simulink model "bms_can_pack"  (R2026b)
settings: Solver=VariableStepAuto
undefined symbols (not defined in the file or in its folder): Ts
libraries: svdutilitieslib x7, simulink x1
settings Model: Creator=aomar  LastModifiedBy=aomar

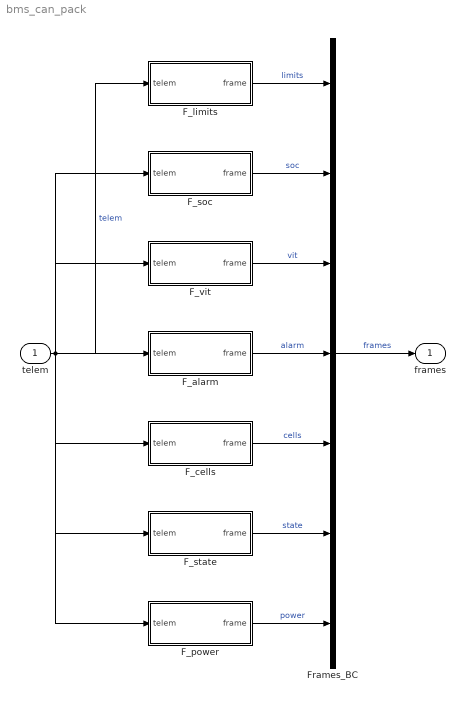
== system bms_can_pack ==
  telem : Inport  OutDataTypeStr=Bus: Bus_BMS_Telemetry  SampleTime=Ts.hk
  F_alarm : Subsystem
  F_cells : Subsystem
  F_limits : Subsystem
  F_power : Subsystem
  F_soc : Subsystem
  F_state : Subsystem
  F_vit : Subsystem
  Frames_BC : BusCreator  Inputs=7  OutDataTypeStr=Bus: Bus_Can1_Bms  NonVirtualBus=on
      settings: InheritFromInputs=off
  frames : Outport  OutDataTypeStr=Bus: Bus_Can1_Bms
  wires:
  telem/1 -> F_limits/1(telem), F_power/1(telem), F_soc/1(telem), F_state/1(telem), F_vit/1(telem), F_cells/1(telem), F_alarm/1(telem)  "telem"
  F_limits/1(frame) -> Frames_BC/1  "limits"
  F_soc/1(frame) -> Frames_BC/2  "soc"
  F_vit/1(frame) -> Frames_BC/3  "vit"
  F_alarm/1(frame) -> Frames_BC/4  "alarm"
  F_cells/1(frame) -> Frames_BC/5  "cells"
  F_state/1(frame) -> Frames_BC/6  "state"
  F_power/1(frame) -> Frames_BC/7  "power"
  Frames_BC/1 -> frames/1  "frames"

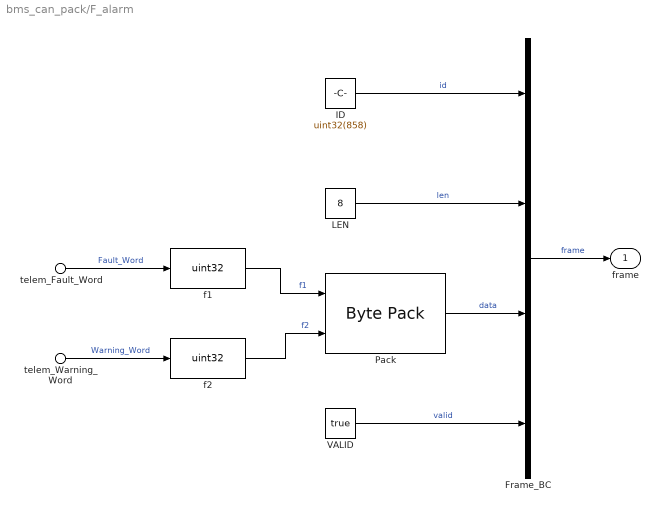
== system bms_can_pack/F_alarm ==
  telem_Fault_Word : Inport  PortName=telem  Element=Fault_Word
  telem_Warning_Word : Inport  PortName=telem  Element=Warning_Word
  Frame_BC : BusCreator  Inputs=4  OutDataTypeStr=Bus: Bus_CanFrame8  NonVirtualBus=on
      settings: InheritFromInputs=off
  ID : Constant  Value=uint32(858)  OutDataTypeStr=uint32  SampleTime=Ts.hk
  LEN : Constant  Value=8  OutDataTypeStr=uint8  SampleTime=Ts.hk
  Pack : svdutilitieslib/Byte Pack  maskPackedDataType=uint8  datatypes={'uint32','uint32'}  byteAlign=1  blockPlatform=arduinoert
      settings: LibrarySourceBlock=mcblib/Signal Management/Byte Pack
  VALID : Constant  Value=true  OutDataTypeStr=boolean  SampleTime=Ts.hk
  f1 : DataTypeConversion  OutDataTypeStr=uint32  RndMeth=Nearest
  f2 : DataTypeConversion  OutDataTypeStr=uint32  RndMeth=Nearest
  frame : Outport  OutDataTypeStr=Bus: Bus_CanFrame8
  wires:
  telem_Fault_Word/1 -> f1/1  "Fault_Word"
  telem_Warning_Word/1 -> f2/1  "Warning_Word"
  f1/1 -> Pack/1  "f1"
  f2/1 -> Pack/2  "f2"
  ID/1 -> Frame_BC/1  "id"
  LEN/1 -> Frame_BC/2  "len"
  VALID/1 -> Frame_BC/4  "valid"
  Pack/1 -> Frame_BC/3  "data"
  Frame_BC/1 -> frame/1  "frame"

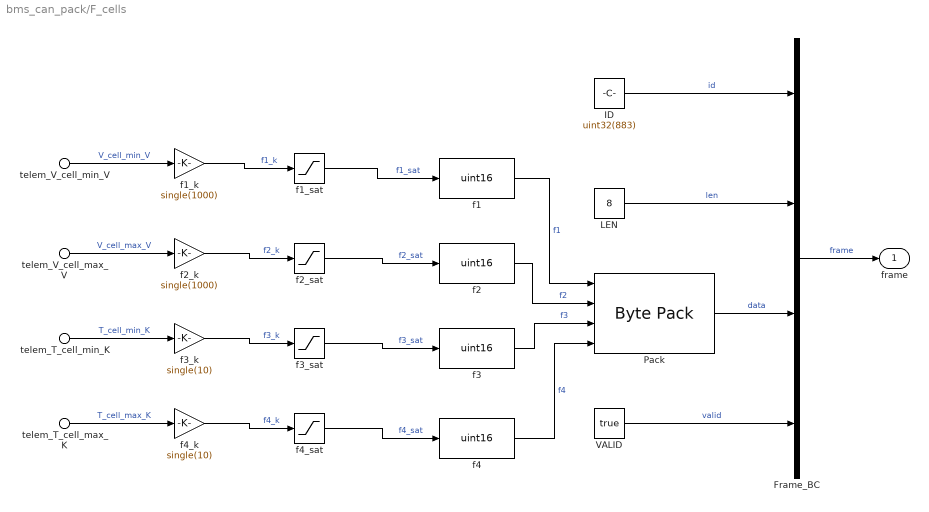
== system bms_can_pack/F_cells ==
  telem_V_cell_min_V : Inport  PortName=telem  Element=V_cell_min_V
  telem_V_cell_max_V : Inport  PortName=telem  Element=V_cell_max_V
  telem_T_cell_min_K : Inport  PortName=telem  Element=T_cell_min_K
  telem_T_cell_max_K : Inport  PortName=telem  Element=T_cell_max_K
  Frame_BC : BusCreator  Inputs=4  OutDataTypeStr=Bus: Bus_CanFrame8  NonVirtualBus=on
      settings: InheritFromInputs=off
  ID : Constant  Value=uint32(883)  OutDataTypeStr=uint32  SampleTime=Ts.hk
  LEN : Constant  Value=8  OutDataTypeStr=uint8  SampleTime=Ts.hk
  Pack : svdutilitieslib/Byte Pack  maskPackedDataType=uint8  datatypes={'uint16','uint16','uint16','uint16'}  byteAlign=1  blockPlatform=arduinoert
      settings: LibrarySourceBlock=mcblib/Signal Management/Byte Pack
  VALID : Constant  Value=true  OutDataTypeStr=boolean  SampleTime=Ts.hk
  f{1..4} (4 alike) : DataTypeConversion  OutDataTypeStr=uint16  RndMeth=Nearest
  f1_k : Gain  Gain=single(1000)
  f1_sat : Saturate  UpperLimit=single(intmax('uint16'))  LowerLimit=single(intmin('uint16'))
  f2_k : Gain  Gain=single(1000)
  f2_sat : Saturate  UpperLimit=single(intmax('uint16'))  LowerLimit=single(intmin('uint16'))
  f3_k : Gain  Gain=single(10)
  f3_sat : Saturate  UpperLimit=single(intmax('uint16'))  LowerLimit=single(intmin('uint16'))
  f4_k : Gain  Gain=single(10)
  f4_sat : Saturate  UpperLimit=single(intmax('uint16'))  LowerLimit=single(intmin('uint16'))
  frame : Outport  OutDataTypeStr=Bus: Bus_CanFrame8
  wires:
  telem_V_cell_min_V/1 -> f1_k/1  "V_cell_min_V"
  telem_V_cell_max_V/1 -> f2_k/1  "V_cell_max_V"
  telem_T_cell_min_K/1 -> f3_k/1  "T_cell_min_K"
  telem_T_cell_max_K/1 -> f4_k/1  "T_cell_max_K"
  f1_k/1 -> f1_sat/1  "f1_k"
  f2_k/1 -> f2_sat/1  "f2_k"
  f3_k/1 -> f3_sat/1  "f3_k"
  f4_k/1 -> f4_sat/1  "f4_k"
  f1_sat/1 -> f1/1  "f1_sat"
  f2_sat/1 -> f2/1  "f2_sat"
  f3_sat/1 -> f3/1  "f3_sat"
  f4_sat/1 -> f4/1  "f4_sat"
  f1/1 -> Pack/1  "f1"
  f2/1 -> Pack/2  "f2"
  f3/1 -> Pack/3  "f3"
  f4/1 -> Pack/4  "f4"
  ID/1 -> Frame_BC/1  "id"
  LEN/1 -> Frame_BC/2  "len"
  VALID/1 -> Frame_BC/4  "valid"
  Pack/1 -> Frame_BC/3  "data"
  Frame_BC/1 -> frame/1  "frame"

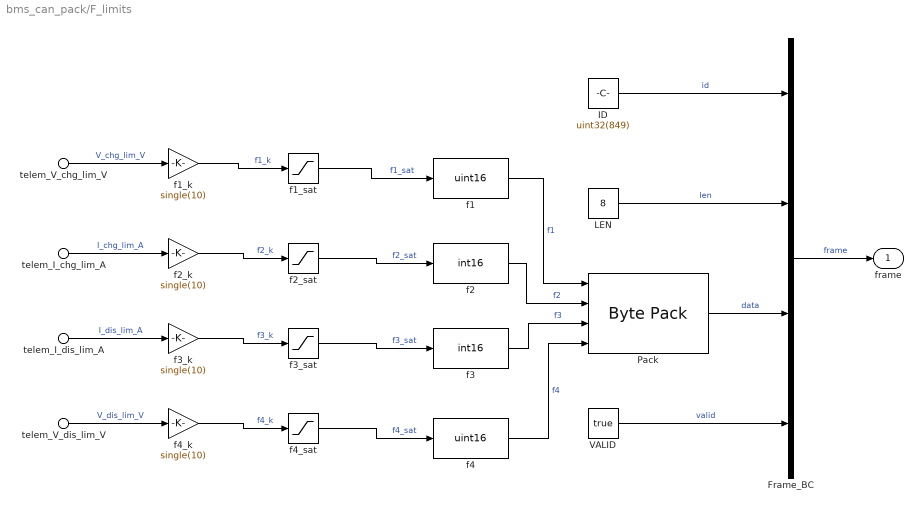
== system bms_can_pack/F_limits ==
  telem_V_chg_lim_V : Inport  PortName=telem  Element=V_chg_lim_V
  telem_I_chg_lim_A : Inport  PortName=telem  Element=I_chg_lim_A
  telem_I_dis_lim_A : Inport  PortName=telem  Element=I_dis_lim_A
  telem_V_dis_lim_V : Inport  PortName=telem  Element=V_dis_lim_V
  Frame_BC : BusCreator  Inputs=4  OutDataTypeStr=Bus: Bus_CanFrame8  NonVirtualBus=on
      settings: InheritFromInputs=off
  ID : Constant  Value=uint32(849)  OutDataTypeStr=uint32  SampleTime=Ts.hk
  LEN : Constant  Value=8  OutDataTypeStr=uint8  SampleTime=Ts.hk
  Pack : svdutilitieslib/Byte Pack  maskPackedDataType=uint8  datatypes={'uint16','int16','int16','uint16'}  byteAlign=1  blockPlatform=arduinoert
      settings: LibrarySourceBlock=mcblib/Signal Management/Byte Pack
  VALID : Constant  Value=true  OutDataTypeStr=boolean  SampleTime=Ts.hk
  f1 : DataTypeConversion  OutDataTypeStr=uint16  RndMeth=Nearest
  f1_k : Gain  Gain=single(10)
  f1_sat : Saturate  UpperLimit=single(intmax('uint16'))  LowerLimit=single(intmin('uint16'))
  f2 : DataTypeConversion  OutDataTypeStr=int16  RndMeth=Nearest
  f2_k : Gain  Gain=single(10)
  f2_sat : Saturate  UpperLimit=single(intmax('int16'))  LowerLimit=single(intmin('int16'))
  f3 : DataTypeConversion  OutDataTypeStr=int16  RndMeth=Nearest
  f3_k : Gain  Gain=single(10)
  f3_sat : Saturate  UpperLimit=single(intmax('int16'))  LowerLimit=single(intmin('int16'))
  f4 : DataTypeConversion  OutDataTypeStr=uint16  RndMeth=Nearest
  f4_k : Gain  Gain=single(10)
  f4_sat : Saturate  UpperLimit=single(intmax('uint16'))  LowerLimit=single(intmin('uint16'))
  frame : Outport  OutDataTypeStr=Bus: Bus_CanFrame8
  wires:
  telem_V_chg_lim_V/1 -> f1_k/1  "V_chg_lim_V"
  telem_I_chg_lim_A/1 -> f2_k/1  "I_chg_lim_A"
  telem_I_dis_lim_A/1 -> f3_k/1  "I_dis_lim_A"
  telem_V_dis_lim_V/1 -> f4_k/1  "V_dis_lim_V"
  f1_k/1 -> f1_sat/1  "f1_k"
  f2_k/1 -> f2_sat/1  "f2_k"
  f3_k/1 -> f3_sat/1  "f3_k"
  f4_k/1 -> f4_sat/1  "f4_k"
  f1_sat/1 -> f1/1  "f1_sat"
  f2_sat/1 -> f2/1  "f2_sat"
  f3_sat/1 -> f3/1  "f3_sat"
  f4_sat/1 -> f4/1  "f4_sat"
  f1/1 -> Pack/1  "f1"
  f2/1 -> Pack/2  "f2"
  f3/1 -> Pack/3  "f3"
  f4/1 -> Pack/4  "f4"
  ID/1 -> Frame_BC/1  "id"
  LEN/1 -> Frame_BC/2  "len"
  VALID/1 -> Frame_BC/4  "valid"
  Pack/1 -> Frame_BC/3  "data"
  Frame_BC/1 -> frame/1  "frame"

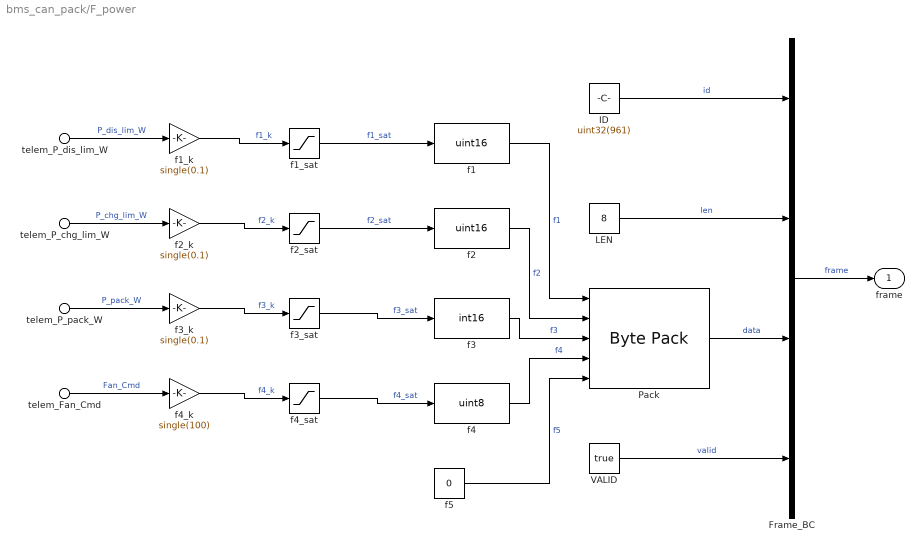
== system bms_can_pack/F_power ==
  telem_P_dis_lim_W : Inport  PortName=telem  Element=P_dis_lim_W
  telem_P_chg_lim_W : Inport  PortName=telem  Element=P_chg_lim_W
  telem_P_pack_W : Inport  PortName=telem  Element=P_pack_W
  telem_Fan_Cmd : Inport  PortName=telem  Element=Fan_Cmd
  Frame_BC : BusCreator  Inputs=4  OutDataTypeStr=Bus: Bus_CanFrame8  NonVirtualBus=on
      settings: InheritFromInputs=off
  ID : Constant  Value=uint32(961)  OutDataTypeStr=uint32  SampleTime=Ts.hk
  LEN : Constant  Value=8  OutDataTypeStr=uint8  SampleTime=Ts.hk
  Pack : svdutilitieslib/Byte Pack  maskPackedDataType=uint8  datatypes={'uint16','uint16','int16','uint8','uint8'}  byteAlign=1  blockPlatform=arduinoert
      settings: LibrarySourceBlock=mcblib/Signal Management/Byte Pack
  VALID : Constant  Value=true  OutDataTypeStr=boolean  SampleTime=Ts.hk
  f1 : DataTypeConversion  OutDataTypeStr=uint16  RndMeth=Nearest
  f1_k : Gain  Gain=single(0.1)
  f1_sat : Saturate  UpperLimit=single(intmax('uint16'))  LowerLimit=single(intmin('uint16'))
  f2 : DataTypeConversion  OutDataTypeStr=uint16  RndMeth=Nearest
  f2_k : Gain  Gain=single(0.1)
  f2_sat : Saturate  UpperLimit=single(intmax('uint16'))  LowerLimit=single(intmin('uint16'))
  f3 : DataTypeConversion  OutDataTypeStr=int16  RndMeth=Nearest
  f3_k : Gain  Gain=single(0.1)
  f3_sat : Saturate  UpperLimit=single(intmax('int16'))  LowerLimit=single(intmin('int16'))
  f4 : DataTypeConversion  OutDataTypeStr=uint8  RndMeth=Nearest
  f4_k : Gain  Gain=single(100)
  f4_sat : Saturate  UpperLimit=single(intmax('uint8'))  LowerLimit=single(intmin('uint8'))
  f5 : Constant  Value=0  OutDataTypeStr=uint8  SampleTime=Ts.hk
  frame : Outport  OutDataTypeStr=Bus: Bus_CanFrame8
  wires:
  telem_P_dis_lim_W/1 -> f1_k/1  "P_dis_lim_W"
  telem_P_chg_lim_W/1 -> f2_k/1  "P_chg_lim_W"
  telem_P_pack_W/1 -> f3_k/1  "P_pack_W"
  telem_Fan_Cmd/1 -> f4_k/1  "Fan_Cmd"
  f1_k/1 -> f1_sat/1  "f1_k"
  f2_k/1 -> f2_sat/1  "f2_k"
  f3_k/1 -> f3_sat/1  "f3_k"
  f4_k/1 -> f4_sat/1  "f4_k"
  f1_sat/1 -> f1/1  "f1_sat"
  f2_sat/1 -> f2/1  "f2_sat"
  f3_sat/1 -> f3/1  "f3_sat"
  f4_sat/1 -> f4/1  "f4_sat"
  f5/1 -> Pack/5  "f5"
  f1/1 -> Pack/1  "f1"
  f2/1 -> Pack/2  "f2"
  f3/1 -> Pack/3  "f3"
  f4/1 -> Pack/4  "f4"
  ID/1 -> Frame_BC/1  "id"
  LEN/1 -> Frame_BC/2  "len"
  VALID/1 -> Frame_BC/4  "valid"
  Pack/1 -> Frame_BC/3  "data"
  Frame_BC/1 -> frame/1  "frame"

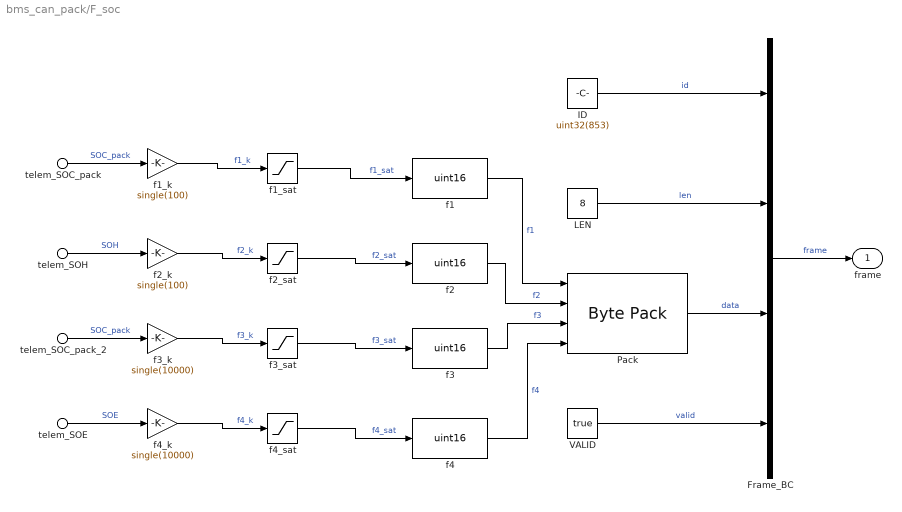
== system bms_can_pack/F_soc ==
  telem_SOC_pack : Inport  PortName=telem  Element=SOC_pack
  telem_SOC_pack_2 : Inport  PortName=telem  Element=SOC_pack
  telem_SOH : Inport  PortName=telem  Element=SOH
  telem_SOE : Inport  PortName=telem  Element=SOE
  Frame_BC : BusCreator  Inputs=4  OutDataTypeStr=Bus: Bus_CanFrame8  NonVirtualBus=on
      settings: InheritFromInputs=off
  ID : Constant  Value=uint32(853)  OutDataTypeStr=uint32  SampleTime=Ts.hk
  LEN : Constant  Value=8  OutDataTypeStr=uint8  SampleTime=Ts.hk
  Pack : svdutilitieslib/Byte Pack  maskPackedDataType=uint8  datatypes={'uint16','uint16','uint16','uint16'}  byteAlign=1  blockPlatform=arduinoert
      settings: LibrarySourceBlock=mcblib/Signal Management/Byte Pack
  VALID : Constant  Value=true  OutDataTypeStr=boolean  SampleTime=Ts.hk
  f{1..4} (4 alike) : DataTypeConversion  OutDataTypeStr=uint16  RndMeth=Nearest
  f1_k : Gain  Gain=single(100)
  f1_sat : Saturate  UpperLimit=single(intmax('uint16'))  LowerLimit=single(intmin('uint16'))
  f2_k : Gain  Gain=single(100)
  f2_sat : Saturate  UpperLimit=single(intmax('uint16'))  LowerLimit=single(intmin('uint16'))
  f3_k : Gain  Gain=single(10000)
  f3_sat : Saturate  UpperLimit=single(intmax('uint16'))  LowerLimit=single(intmin('uint16'))
  f4_k : Gain  Gain=single(10000)
  f4_sat : Saturate  UpperLimit=single(intmax('uint16'))  LowerLimit=single(intmin('uint16'))
  frame : Outport  OutDataTypeStr=Bus: Bus_CanFrame8
  wires:
  telem_SOC_pack/1 -> f1_k/1  "SOC_pack"
  telem_SOH/1 -> f2_k/1  "SOH"
  telem_SOC_pack_2/1 -> f3_k/1  "SOC_pack"
  telem_SOE/1 -> f4_k/1  "SOE"
  f1_k/1 -> f1_sat/1  "f1_k"
  f2_k/1 -> f2_sat/1  "f2_k"
  f3_k/1 -> f3_sat/1  "f3_k"
  f4_k/1 -> f4_sat/1  "f4_k"
  f1_sat/1 -> f1/1  "f1_sat"
  f2_sat/1 -> f2/1  "f2_sat"
  f3_sat/1 -> f3/1  "f3_sat"
  f4_sat/1 -> f4/1  "f4_sat"
  f1/1 -> Pack/1  "f1"
  f2/1 -> Pack/2  "f2"
  f3/1 -> Pack/3  "f3"
  f4/1 -> Pack/4  "f4"
  ID/1 -> Frame_BC/1  "id"
  LEN/1 -> Frame_BC/2  "len"
  VALID/1 -> Frame_BC/4  "valid"
  Pack/1 -> Frame_BC/3  "data"
  Frame_BC/1 -> frame/1  "frame"

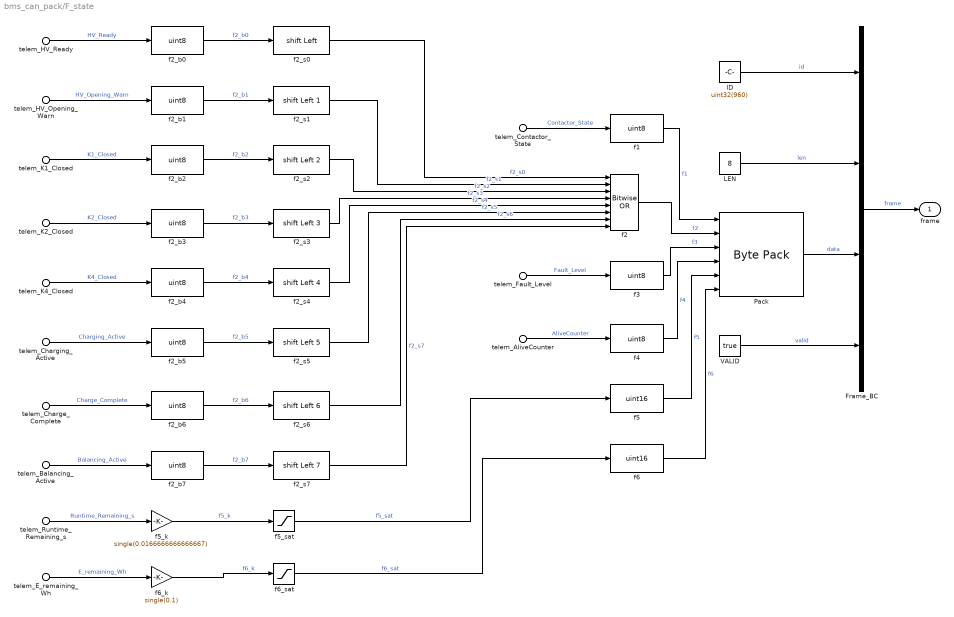
== system bms_can_pack/F_state ==
  telem_Contactor_State : Inport  PortName=telem  Element=Contactor_State
  telem_HV_Ready : Inport  PortName=telem  Element=HV_Ready
  telem_HV_Opening_Warn : Inport  PortName=telem  Element=HV_Opening_Warn
  telem_K1_Closed : Inport  PortName=telem  Element=K1_Closed
  telem_K2_Closed : Inport  PortName=telem  Element=K2_Closed
  telem_K4_Closed : Inport  PortName=telem  Element=K4_Closed
  telem_Charging_Active : Inport  PortName=telem  Element=Charging_Active
  telem_Charge_Complete : Inport  PortName=telem  Element=Charge_Complete
  telem_Balancing_Active : Inport  PortName=telem  Element=Balancing_Active
  telem_Fault_Level : Inport  PortName=telem  Element=Fault_Level
  telem_AliveCounter : Inport  PortName=telem  Element=AliveCounter
  telem_Runtime_Remaining_s : Inport  PortName=telem  Element=Runtime_Remaining_s
  telem_E_remaining_Wh : Inport  PortName=telem  Element=E_remaining_Wh
  Frame_BC : BusCreator  Inputs=4  OutDataTypeStr=Bus: Bus_CanFrame8  NonVirtualBus=on
      settings: InheritFromInputs=off
  ID : Constant  Value=uint32(960)  OutDataTypeStr=uint32  SampleTime=Ts.hk
  LEN : Constant  Value=8  OutDataTypeStr=uint8  SampleTime=Ts.hk
  Pack : svdutilitieslib/Byte Pack  maskPackedDataType=uint8  datatypes={'uint8','uint8','uint8','uint8','uint16','uint16'}  byteAlign=1  blockPlatform=arduinoert
      settings: LibrarySourceBlock=mcblib/Signal Management/Byte Pack
  VALID : Constant  Value=true  OutDataTypeStr=boolean  SampleTime=Ts.hk
  f1 : DataTypeConversion  OutDataTypeStr=uint8  RndMeth=Nearest
  f2 : simulink/Logic and Bit Operations/Bitwise Operator  logicop=OR  UseBitMask=off  NumInputPorts=8  BitMask=bin2dec('11011001')  BitMaskRealWorld=Stored Integer
  f2_b{0..7} (8 alike) : DataTypeConversion  OutDataTypeStr=uint8  RndMeth=Nearest
  f2_s0 : ArithShift  BitShiftDirection=Left
  f2_s1 : ArithShift  BitShiftNumber=1  BitShiftDirection=Left
  f2_s2 : ArithShift  BitShiftNumber=2  BitShiftDirection=Left
  f2_s3 : ArithShift  BitShiftNumber=3  BitShiftDirection=Left
  f2_s4 : ArithShift  BitShiftNumber=4  BitShiftDirection=Left
  f2_s5 : ArithShift  BitShiftNumber=5  BitShiftDirection=Left
  f2_s6 : ArithShift  BitShiftNumber=6  BitShiftDirection=Left
  f2_s7 : ArithShift  BitShiftNumber=7  BitShiftDirection=Left
  f3 : DataTypeConversion  OutDataTypeStr=uint8  RndMeth=Nearest
  f4 : DataTypeConversion  OutDataTypeStr=uint8  RndMeth=Nearest
  f5 : DataTypeConversion  OutDataTypeStr=uint16  RndMeth=Nearest
  f5_k : Gain  Gain=single(0.0166666666666667)
  f5_sat : Saturate  UpperLimit=single(intmax('uint16'))  LowerLimit=single(intmin('uint16'))
  f6 : DataTypeConversion  OutDataTypeStr=uint16  RndMeth=Nearest
  f6_k : Gain  Gain=single(0.1)
  f6_sat : Saturate  UpperLimit=single(intmax('uint16'))  LowerLimit=single(intmin('uint16'))
  frame : Outport  OutDataTypeStr=Bus: Bus_CanFrame8
  wires:
  telem_HV_Ready/1 -> f2_b0/1  "HV_Ready"
  telem_HV_Opening_Warn/1 -> f2_b1/1  "HV_Opening_Warn"
  telem_K1_Closed/1 -> f2_b2/1  "K1_Closed"
  telem_K2_Closed/1 -> f2_b3/1  "K2_Closed"
  telem_K4_Closed/1 -> f2_b4/1  "K4_Closed"
  telem_Charging_Active/1 -> f2_b5/1  "Charging_Active"
  telem_Charge_Complete/1 -> f2_b6/1  "Charge_Complete"
  telem_Balancing_Active/1 -> f2_b7/1  "Balancing_Active"
  telem_Runtime_Remaining_s/1 -> f5_k/1  "Runtime_Remaining_s"
  telem_E_remaining_Wh/1 -> f6_k/1  "E_remaining_Wh"
  f5_k/1 -> f5_sat/1  "f5_k"
  f6_k/1 -> f6_sat/1  "f6_k"
  f2_b0/1 -> f2_s0/1  "f2_b0"
  f2_b1/1 -> f2_s1/1  "f2_b1"
  f2_b2/1 -> f2_s2/1  "f2_b2"
  f2_b3/1 -> f2_s3/1  "f2_b3"
  f2_b4/1 -> f2_s4/1  "f2_b4"
  f2_b5/1 -> f2_s5/1  "f2_b5"
  f2_b6/1 -> f2_s6/1  "f2_b6"
  f2_b7/1 -> f2_s7/1  "f2_b7"
  f5_sat/1 -> f5/1  "f5_sat"
  f6_sat/1 -> f6/1  "f6_sat"
  f2_s0/1 -> f2/1  "f2_s0"
  f2_s1/1 -> f2/2  "f2_s1"
  f2_s2/1 -> f2/3  "f2_s2"
  f2_s3/1 -> f2/4  "f2_s3"
  f2_s4/1 -> f2/5  "f2_s4"
  f2_s5/1 -> f2/6  "f2_s5"
  f2_s6/1 -> f2/7  "f2_s6"
  f2_s7/1 -> f2/8  "f2_s7"
  telem_Contactor_State/1 -> f1/1  "Contactor_State"
  telem_Fault_Level/1 -> f3/1  "Fault_Level"
  telem_AliveCounter/1 -> f4/1  "AliveCounter"
  f2/1 -> Pack/2  "f2"
  f1/1 -> Pack/1  "f1"
  f3/1 -> Pack/3  "f3"
  f4/1 -> Pack/4  "f4"
  f5/1 -> Pack/5  "f5"
  f6/1 -> Pack/6  "f6"
  ID/1 -> Frame_BC/1  "id"
  LEN/1 -> Frame_BC/2  "len"
  VALID/1 -> Frame_BC/4  "valid"
  Pack/1 -> Frame_BC/3  "data"
  Frame_BC/1 -> frame/1  "frame"

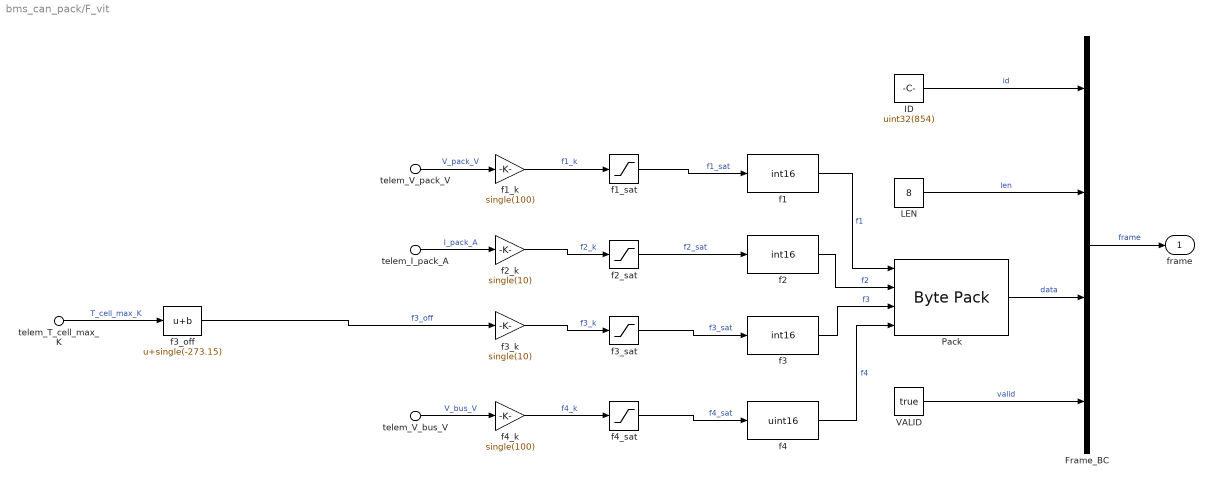
== system bms_can_pack/F_vit ==
  telem_V_pack_V : Inport  PortName=telem  Element=V_pack_V
  telem_I_pack_A : Inport  PortName=telem  Element=I_pack_A
  telem_T_cell_max_K : Inport  PortName=telem  Element=T_cell_max_K
  telem_V_bus_V : Inport  PortName=telem  Element=V_bus_V
  Frame_BC : BusCreator  Inputs=4  OutDataTypeStr=Bus: Bus_CanFrame8  NonVirtualBus=on
      settings: InheritFromInputs=off
  ID : Constant  Value=uint32(854)  OutDataTypeStr=uint32  SampleTime=Ts.hk
  LEN : Constant  Value=8  OutDataTypeStr=uint8  SampleTime=Ts.hk
  Pack : svdutilitieslib/Byte Pack  maskPackedDataType=uint8  datatypes={'int16','int16','int16','uint16'}  byteAlign=1  blockPlatform=arduinoert
      settings: LibrarySourceBlock=mcblib/Signal Management/Byte Pack
  VALID : Constant  Value=true  OutDataTypeStr=boolean  SampleTime=Ts.hk
  f1 : DataTypeConversion  OutDataTypeStr=int16  RndMeth=Nearest
  f1_k : Gain  Gain=single(100)
  f1_sat : Saturate  UpperLimit=single(intmax('int16'))  LowerLimit=single(intmin('int16'))
  f2 : DataTypeConversion  OutDataTypeStr=int16  RndMeth=Nearest
  f2_k : Gain  Gain=single(10)
  f2_sat : Saturate  UpperLimit=single(intmax('int16'))  LowerLimit=single(intmin('int16'))
  f3 : DataTypeConversion  OutDataTypeStr=int16  RndMeth=Nearest
  f3_k : Gain  Gain=single(10)
  f3_off : Bias  Bias=single(-273.15)  SaturateOnIntegerOverflow=off
  f3_sat : Saturate  UpperLimit=single(intmax('int16'))  LowerLimit=single(intmin('int16'))
  f4 : DataTypeConversion  OutDataTypeStr=uint16  RndMeth=Nearest
  f4_k : Gain  Gain=single(100)
  f4_sat : Saturate  UpperLimit=single(intmax('uint16'))  LowerLimit=single(intmin('uint16'))
  frame : Outport  OutDataTypeStr=Bus: Bus_CanFrame8
  wires:
  telem_T_cell_max_K/1 -> f3_off/1  "T_cell_max_K"
  f3_off/1 -> f3_k/1  "f3_off"
  telem_V_pack_V/1 -> f1_k/1  "V_pack_V"
  telem_I_pack_A/1 -> f2_k/1  "I_pack_A"
  telem_V_bus_V/1 -> f4_k/1  "V_bus_V"
  f1_k/1 -> f1_sat/1  "f1_k"
  f2_k/1 -> f2_sat/1  "f2_k"
  f3_k/1 -> f3_sat/1  "f3_k"
  f4_k/1 -> f4_sat/1  "f4_k"
  f1_sat/1 -> f1/1  "f1_sat"
  f2_sat/1 -> f2/1  "f2_sat"
  f3_sat/1 -> f3/1  "f3_sat"
  f4_sat/1 -> f4/1  "f4_sat"
  f1/1 -> Pack/1  "f1"
  f2/1 -> Pack/2  "f2"
  f3/1 -> Pack/3  "f3"
  f4/1 -> Pack/4  "f4"
  ID/1 -> Frame_BC/1  "id"
  LEN/1 -> Frame_BC/2  "len"
  VALID/1 -> Frame_BC/4  "valid"
  Pack/1 -> Frame_BC/3  "data"
  Frame_BC/1 -> frame/1  "frame"
